simulink model "NanoBalancer_Stabilizer"  (R2026b)
settings: Solver=ode45  StopTime=4  MaxStep=1e-3  RelTol=1e-6
PreLoadFcn:
  | InitNanoBalancer
InitFcn:
  | InitNanoBalancer
values from neighbouring files (symbols this model uses):
  bump_dt = 0.02    [check_predictor.m]    (also in run_NanoBalancer_Encoder.m; run_NanoBalancer_Stabilizer.m)
  bump_t = 1    [check_predictor.m]    (also in run_NanoBalancer_Encoder.m; run_NanoBalancer_Stabilizer.m)
  FrictionComp = 1    [run_NanoBalancer_Encoder.m]
  sampleTime = NB.Ts    [InitNanoBalancer.m]
  SensorMode = m; InitNanoBalancer    [check_predictor.m]    (also in run_NanoBalancer_Encoder.m = runs{k,2}; run_NanoBalancer_Stabilizer.m)
  x0 = [deg2rad(theta0_deg); 0; 0; 0]    [InitNanoBalancer.m]
undefined symbols (not defined in the file or in its folder): NB
settings Model: Creator=arkad  LastModifiedBy=arkad

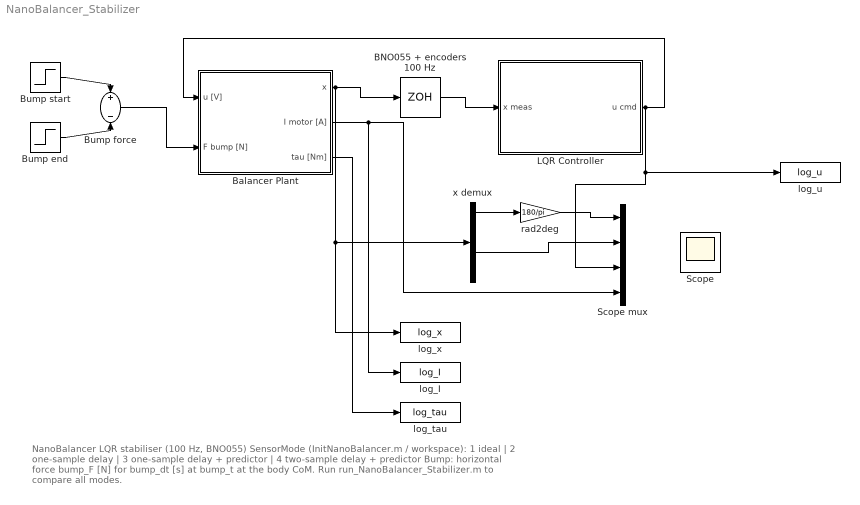
== system NanoBalancer_Stabilizer ==
  note: NanoBalancer LQR stabiliser (100 Hz, BNO055)
      | SensorMode (InitNanoBalancer.m / workspace): 1 ideal | 2 one-sample delay | 3 one-sample delay + predictor | 4 two-sample delay + predictor
      | Bump: horizontal force bump_F [N] for bump_dt [s] at bump_t at the body CoM.
      | Run run_NanoBalancer_Stabilizer.m to compare all modes.
  BNO055 + encoders 100 Hz : ZeroOrderHold  SampleTime=sampleTime
  Balancer Plant : Subsystem
  Bump end : Step  Time=bump_t+bump_dt  FinalValue=bump_F  SampleTime=0
  Bump force : Sum  Inputs=+-
  Bump start : Step  Time=bump_t  FinalValue=bump_F  SampleTime=0
  LQR Controller : Subsystem
  Scope : Scope
  Scope mux : Mux
  log_I : ToWorkspace  VariableName=log_I  SaveFormat=Structure With Time  SampleTime=-1
  log_tau : ToWorkspace  VariableName=log_tau  SaveFormat=Structure With Time  SampleTime=-1
  log_u : ToWorkspace  VariableName=log_u  SaveFormat=Structure With Time  SampleTime=-1
  log_x : ToWorkspace  VariableName=log_x  SaveFormat=Structure With Time  SampleTime=-1
  rad2deg : Gain  Gain=180/pi
  x demux : Demux
  wires:
  Bump start/1 -> Bump force/1
  Bump end/1 -> Bump force/2
  Bump force/1 -> Balancer Plant/2(F bump [N])
  Balancer Plant/1(x) -> x demux/1, log_x/1, BNO055 + encoders 100 Hz/1
  BNO055 + encoders 100 Hz/1 -> LQR Controller/1(x meas)
  LQR Controller/1(u cmd) -> Scope mux/3, log_u/1, Balancer Plant/1(u [V])
  x demux/1 -> rad2deg/1
  rad2deg/1 -> Scope mux/1
  x demux/3 -> Scope mux/2
  Balancer Plant/2(I motor [A]) -> Scope mux/4, log_I/1
  Balancer Plant/3(tau [Nm]) -> log_tau/1

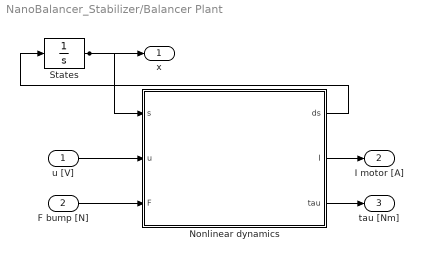
== system NanoBalancer_Stabilizer/Balancer Plant ==
  u [V] : Inport
  F bump [N] : Inport  Port=2
  Nonlinear dynamics : MATLAB Function  TreatAsAtomicUnit=on
  States : Integrator  InitialCondition=x0
  x : Outport
  I motor [A] : Outport  Port=2
  tau [Nm] : Outport  Port=3
  wires:
  States/1 -> Nonlinear dynamics/1(s), x/1
  Nonlinear dynamics/3(tau) -> tau [Nm]/1
  Nonlinear dynamics/2(I) -> I motor [A]/1
  F bump [N]/1 -> Nonlinear dynamics/3(F)
  u [V]/1 -> Nonlinear dynamics/2(u)
  Nonlinear dynamics/1(ds) -> States/1

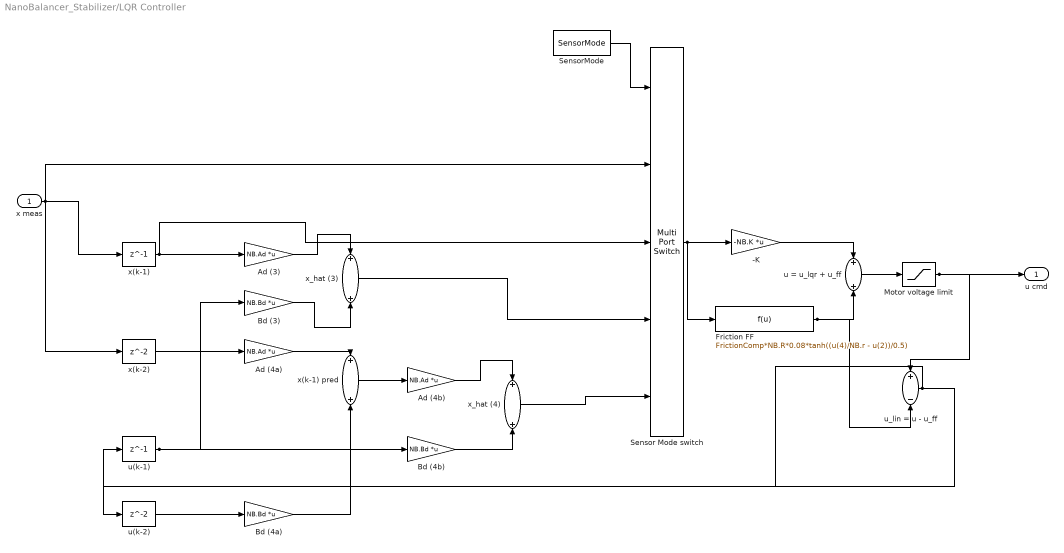
== system NanoBalancer_Stabilizer/LQR Controller ==
  x meas : Inport
  -K : Gain  Gain=-NB.K  Multiplication=Matrix(K*u)
  Ad (3) : Gain  Gain=NB.Ad  Multiplication=Matrix(K*u)
  Ad (4a) : Gain  Gain=NB.Ad  Multiplication=Matrix(K*u)
  Ad (4b) : Gain  Gain=NB.Ad  Multiplication=Matrix(K*u)
  Bd (3) : Gain  Gain=NB.Bd  Multiplication=Matrix(K*u)
  Bd (4a) : Gain  Gain=NB.Bd  Multiplication=Matrix(K*u)
  Bd (4b) : Gain  Gain=NB.Bd  Multiplication=Matrix(K*u)
  Friction FF : Fcn  Expr=FrictionComp*NB.R*0.08*tanh((u(4)/NB.r - u(2))/0.5)
  Motor voltage limit : Saturate  UpperLimit=NB.Vmax  LowerLimit=-NB.Vmax
  Sensor Mode switch : MultiPortSwitch  Inputs=4  SaturateOnIntegerOverflow=off  InputSameDT=off
  SensorMode : Constant  Value=SensorMode
  u = u_lqr + u_ff : Sum
  u(k-1) : Delay  DelayLength=1  InitialCondition=0  SampleTime=sampleTime
  u(k-2) : Delay  InitialCondition=0  SampleTime=sampleTime
  u_lin = u - u_ff : Sum  Inputs=+-
  x(k-1) : Delay  DelayLength=1  InitialCondition=0  SampleTime=sampleTime
  x(k-1) pred : Sum
  x(k-2) : Delay  InitialCondition=0  SampleTime=sampleTime
  x_hat (3) : Sum
  x_hat (4) : Sum
  u cmd : Outport
  wires:
  x meas/1 -> x(k-1)/1, x(k-2)/1, Sensor Mode switch/2
  x(k-1)/1 -> Ad (3)/1, Sensor Mode switch/3
  u(k-1)/1 -> Bd (3)/1, Bd (4b)/1
  Ad (3)/1 -> x_hat (3)/1
  Bd (3)/1 -> x_hat (3)/2
  x(k-2)/1 -> Ad (4a)/1
  u(k-2)/1 -> Bd (4a)/1
  Ad (4a)/1 -> x(k-1) pred/1
  Bd (4a)/1 -> x(k-1) pred/2
  x(k-1) pred/1 -> Ad (4b)/1
  Ad (4b)/1 -> x_hat (4)/1
  Bd (4b)/1 -> x_hat (4)/2
  SensorMode/1 -> Sensor Mode switch/1
  x_hat (3)/1 -> Sensor Mode switch/4
  x_hat (4)/1 -> Sensor Mode switch/5
  Sensor Mode switch/1 -> -K/1, Friction FF/1
  -K/1 -> u = u_lqr + u_ff/1
  Friction FF/1 -> u = u_lqr + u_ff/2, u_lin = u - u_ff/2
  u = u_lqr + u_ff/1 -> Motor voltage limit/1
  Motor voltage limit/1 -> u cmd/1, u_lin = u - u_ff/1
  u_lin = u - u_ff/1 -> u(k-1)/1, u(k-2)/1

== matlab function NanoBalancer_Stabilizer/Balancer Plant/Nonlinear dynamics ==
  data: s input size=[4 1]; u input; ds output; F input; I output; tau output; NB_pp parameter size=[1 12]
function [ds, I, tau] = fcn(s, u, F, NB_pp)
pp = NB_pp;
% Nonlinear wheeled inverted pendulum + DC motor with driver current limit.
% s = [theta; theta_dot; x; x_dot], u = voltage to both motors, F = force at CoM
m_b=pp(1); m_w=pp(2); l=pp(3); Ib=pp(4); Iw=pp(5); r=pp(6); g=pp(7);
Kt=pp(8); Ke=pp(9); R=pp(10); Ilim=pp(11); Inl=pp(12);
th = s(1); thd = s(2); xd = s(4);
wm = xd/r - thd;                         % motor output speed relative to body
I = (u - Ke*wm)/R;
I = min(max(I, -Ilim), Ilim);            % Nano Motor Carrier 0.5 A limit
Tm = Kt*I - Kt*Inl*tanh(wm/0.5);         % per motor, incl. no-load friction
tau = 2*Tm;
a = Ib + m_b*l^2;  b = m_b*r*l;  c = Iw + (m_b + m_w)*r^2;
M = [a, b*cos(th); b*cos(th), c];
f = [m_b*g*l*sin(th) - tau + F*l*cos(th); tau + b*sin(th)*thd^2 + F*r];
acc = M\f;
ds = [thd; acc(1); xd; r*acc(2)];
